simulink model "swift_6dof_sitl"  (R2026a)
settings: Solver=ode4  StopTime=inf  FixedStep=P.sitl.dt  MaxStep=0.01  RelTol=1e-6
InitFcn:
  | if ~evalin('base','exist(''P'',''var'')')
  |     evalin('base','swift_placeholder');
  | end
  | evalin('base','P = swift_sitl_params(P);');
StopFcn:
  | clear ap_json_step
undefined symbols (not defined in the file): P
libraries: aerolibasang x2, aerolibadyn x1, aerolibatmos2 x1
settings Model: Creator=rbilo  LastModifiedBy=Ryan

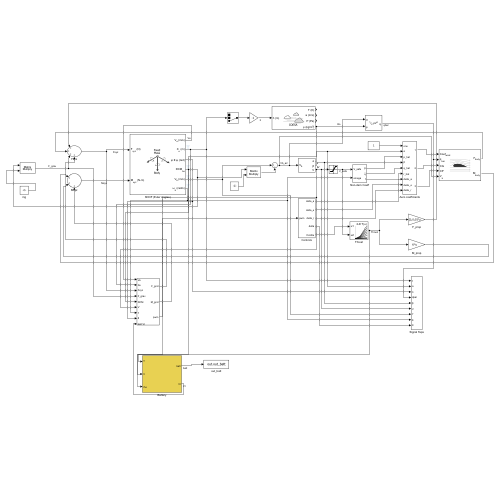
[thumbnail: Simulink's stored preview of the top-level diagram]
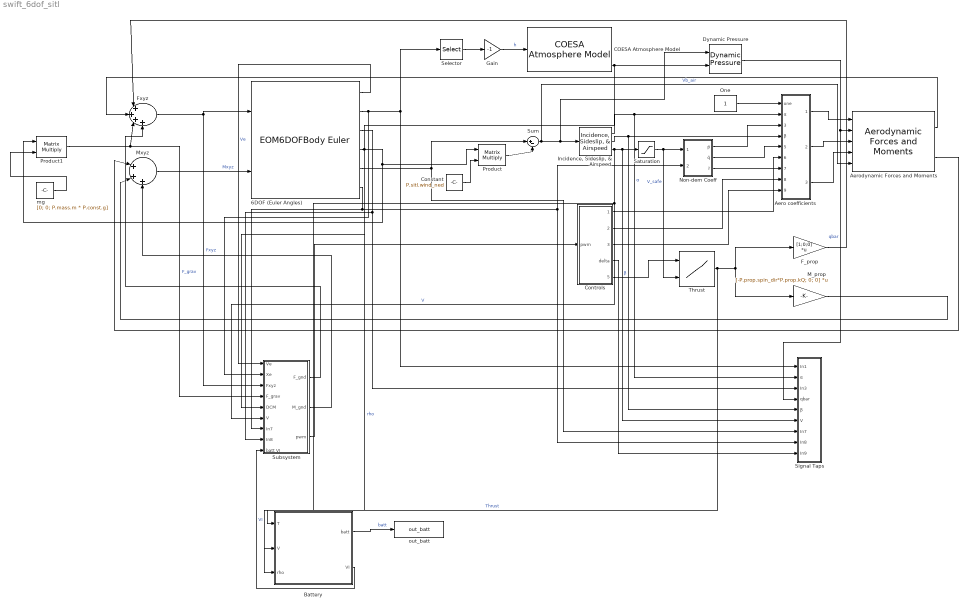
== system swift_6dof_sitl ==
  6DOF (Euler Angles) : EOM6DOFBodyEuler  xme_0=P.sitl.ic.pos0'  Vm_0=P.sitl.ic.uvw0'  eul_0=P.sitl.ic.euler0'  pm_0=P.sitl.ic.om0'  mass_0=P.mass.m  inertia=P.mass.I
  Aero coefficients : Subsystem
  "Aerodynamic Forces and Moments " : aerolibadyn/Aerodynamic Forces and Moments   inputAxes=Wind  outputForceAxes=Body  outputMomentAxes=Body  S=P.geom.S  b=P.geom.b  cbar=P.geom.c
  Battery : Subsystem
  COESA Atmosphere Model : aerolibatmos2/COESA Atmosphere Model  units=Metric (MKS)  spec=1976 COESA-extended U.S. Standard Atmosphere  model=Profile  profile_var=High temperature  profile_percent=1%  profile_alt=5 km (16404 ft)  envelope_var=High temperature  envelope_percent=1%  action=Warning
  Constant : Constant  Value=P.sitl.wind_ned
  Controls : Subsystem
  Dynamic Pressure : aerolibasang/Dynamic Pressure
  F_prop : Gain  Gain=[1;0;0]  Multiplication=Matrix(K*u)
  Fxyz : Sum  Inputs=|++++
  Gain : Gain  Gain=-1
  "Incidence, Sideslip, & Airspeed" : aerolibasang/Incidence, Sideslip, & Airspeed
  M_prop : Gain  Gain=[-P.prop.spin_dir*P.prop.kQ; 0; 0]  Multiplication=Matrix(K*u)
  Mxyz : Sum  Inputs=|+++
  Non-dem Coeff : Subsystem
  One : Constant
  Product : Product  Multiplication=Matrix(*)
  Product1 : Product  Multiplication=Matrix(*)
  Saturation : Saturate  UpperLimit=inf  LowerLimit=0.5
  Selector : Selector  InputPortWidth=3  IndexOptions=Index vector (dialog)  Indices=3  OutputSizes=1
  Signal Taps : Subsystem
  Subsystem : Subsystem
  Sum : Sum  Inputs=|+-
  Thrust : Lookup_n-D  BreakpointsForDimension1=P.prop.throttle_bp  BreakpointsForDimension2=P.prop.V_bp  Table=P.sitl.thrust_map  ExtrapMethod=Clip  InternalRulePriority=Speed  RndMeth=Simplest
      settings: InputPortMap=u0,u1
  mg : Constant  Value=[0; 0; P.mass.m * P.const.g]
  out_batt : ToWorkspace  VariableName=out_batt  SaveFormat=Timeseries  SampleTime=-1
      settings: Decimation=P.sitl.log_decim
  wires:
  6DOF (Euler Angles)/2 -> Subsystem/2(Xe), Signal Taps/1(In1), Selector/1
  6DOF (Euler Angles)/4 -> Subsystem/5(DCM), Product1/1, Product/1
  Constant/1 -> Product/2
  Selector/1 -> Gain/1
  Gain/1 -> COESA Atmosphere Model/1  "h"
  Product/1 -> Sum/2
  Sum/1 -> "Incidence, Sideslip, & Airspeed"/1, Dynamic Pressure/1, "Aerodynamic Forces and Moments "/5  "Vb_air"
  "Incidence, Sideslip, & Airspeed"/3 -> Subsystem/6(V), Battery/2(V), Signal Taps/6(V), Saturation/1  "V"
  COESA Atmosphere Model/4 -> Dynamic Pressure/2, Battery/3(rho)  "rho"
  Saturation/1 -> Thrust/2, Non-dem Coeff/1(V_safe)  "V_safe"
  6DOF (Euler Angles)/6 -> Subsystem/7(In7), Signal Taps/8(In8), Non-dem Coeff/2(omega)
  Dynamic Pressure/1 -> Signal Taps/4(qbar), "Aerodynamic Forces and Moments "/2  "qbar"
  "Incidence, Sideslip, & Airspeed"/1 -> Signal Taps/2(α), Aero coefficients/2(α)  "α"
  "Incidence, Sideslip, & Airspeed"/2 -> Signal Taps/5(β), Aero coefficients/4(β)  "β"
  Aero coefficients/1(Out1) -> "Aerodynamic Forces and Moments "/1
  Aero coefficients/2(Out2) -> "Aerodynamic Forces and Moments "/3
  Aero coefficients/3(Out3) -> "Aerodynamic Forces and Moments "/4
  One/1 -> Aero coefficients/1(one)
  Non-dem Coeff/1(p̂) -> Aero coefficients/3(p_hat)
  Non-dem Coeff/2(q̂) -> Aero coefficients/5(q_hat)
  Non-dem Coeff/3(r̂) -> Aero coefficients/6(r_hat)
  Controls/1(delta_a) -> Aero coefficients/7(delta_a)
  Controls/2(delta_e) -> Aero coefficients/8(delta_e)
  Controls/3(delta_r) -> Aero coefficients/9(delta_r)
  Controls/5(throttle) -> Thrust/1
  Thrust/1 -> F_prop/1, M_prop/1, Battery/1(T)  "Thrust"
  mg/1 -> Product1/2
  Product1/1 -> Subsystem/4(F_grav), Fxyz/3  "F_grav"
  Fxyz/1 -> Subsystem/3(Fxyz), 6DOF (Euler Angles)/1  "Fxyz"
  F_prop/1 -> Fxyz/1
  Mxyz/1 -> 6DOF (Euler Angles)/2  "Mxyz"
  M_prop/1 -> Mxyz/2
  "Aerodynamic Forces and Moments "/1 -> Fxyz/2
  "Aerodynamic Forces and Moments "/2 -> Mxyz/1
  6DOF (Euler Angles)/5 -> Signal Taps/7(In7), Sum/1
  6DOF (Euler Angles)/3 -> Subsystem/8(In8), Signal Taps/3(In3)
  Controls/4(delta) -> Signal Taps/9(In9)
  6DOF (Euler Angles)/1 -> Subsystem/1(Ve)  "Ve"
  Subsystem/1(F_gnd) -> Fxyz/4
  Subsystem/2(M_gnd) -> Mxyz/3
  Subsystem/3(pwm) -> Controls/1(pwm)
  Battery/1(batt) -> out_batt/1  "batt"
  Battery/2(VI) -> Subsystem/9(batt VI)  "VI"

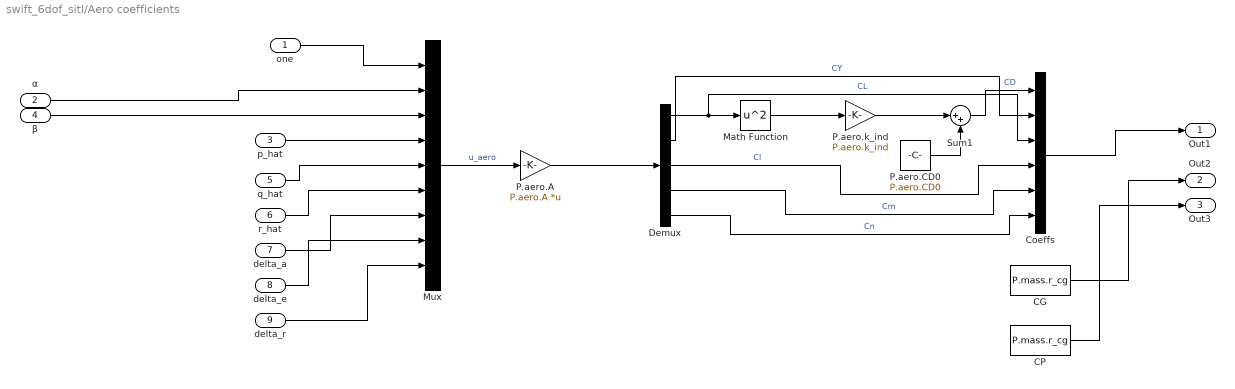
== system swift_6dof_sitl/Aero coefficients ==
  one : Inport
  α : Inport  Port=2
  p_hat : Inport  Port=3
  β : Inport  Port=4
  q_hat : Inport  Port=5
  r_hat : Inport  Port=6
  delta_a : Inport  Port=7
  delta_e : Inport  Port=8
  delta_r : Inport  Port=9
  CG : Constant  Value=P.mass.r_cg
  CP : Constant  Value=P.mass.r_cg
  Coeffs : Mux  Inputs=6
  Demux : Demux  Outputs=5
  Math Function : Math  Operator=square
  Mux : Mux  Inputs=9
  P.aero.A : Gain  Gain=P.aero.A  Multiplication=Matrix(K*u)
  P.aero.CD0 : Constant  Value=P.aero.CD0
  P.aero.k_ind : Gain  Gain=P.aero.k_ind
  Sum1 : Sum  Inputs=|++
  Out1 : Outport
  Out2 : Outport  Port=2
  Out3 : Outport  Port=3
  wires:
  P.aero.CD0/1 -> Sum1/2
  p_hat/1 -> Mux/4
  Demux/1 -> Math Function/1, Coeffs/3  "CL"
  delta_r/1 -> Mux/9
  Math Function/1 -> P.aero.k_ind/1
  CP/1 -> Out3/1
  P.aero.k_ind/1 -> Sum1/1
  P.aero.A/1 -> Demux/1
  delta_a/1 -> Mux/7
  Mux/1 -> P.aero.A/1  "u_aero"
  CG/1 -> Out2/1
  Demux/2 -> Coeffs/2  "CY"
  Sum1/1 -> Coeffs/1  "CD"
  β/1 -> Mux/3
  Demux/5 -> Coeffs/6  "Cn"
  Demux/3 -> Coeffs/4  "Cl"
  Demux/4 -> Coeffs/5  "Cm"
  r_hat/1 -> Mux/6
  Coeffs/1 -> Out1/1
  α/1 -> Mux/2
  q_hat/1 -> Mux/5
  one/1 -> Mux/1
  delta_e/1 -> Mux/8

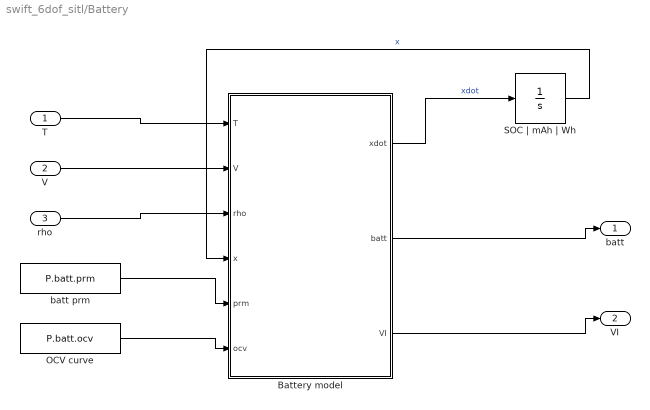
== system swift_6dof_sitl/Battery ==
  T : Inport
  V : Inport  Port=2
  rho : Inport  Port=3
  Battery model : MATLAB Function  TreatAsAtomicUnit=on
  OCV curve : Constant  Value=P.batt.ocv
  SOC | mAh | Wh : Integrator  InitialCondition=P.batt.x0  LimitOutput=on  UpperSaturationLimit=[1; inf; inf]  LowerSaturationLimit=[0; 0; 0]
  batt prm : Constant  Value=P.batt.prm
  batt : Outport
  VI : Outport  Port=2
  wires:
  T/1 -> Battery model/1(T)
  V/1 -> Battery model/2(V)
  rho/1 -> Battery model/3(rho)
  SOC | mAh | Wh/1 -> Battery model/4(x)  "x"
  batt prm/1 -> Battery model/5(prm)
  OCV curve/1 -> Battery model/6(ocv)
  Battery model/1(xdot) -> SOC | mAh | Wh/1  "xdot"
  Battery model/2(batt) -> batt/1
  Battery model/3(VI) -> VI/1

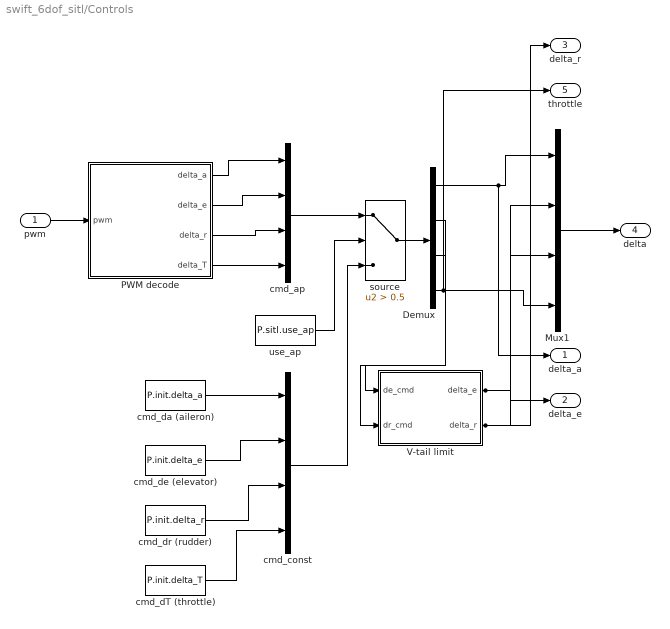
== system swift_6dof_sitl/Controls ==
  pwm : Inport
  Demux : Demux
  Mux1 : Mux
  PWM decode : Subsystem
  V-tail limit : Subsystem
  cmd_ap : Mux
  cmd_const : Mux
  cmd_dT (throttle) : Constant  Value=P.init.delta_T
  cmd_da (aileron) : Constant  Value=P.init.delta_a
  cmd_de (elevator) : Constant  Value=P.init.delta_e
  cmd_dr (rudder) : Constant  Value=P.init.delta_r
  source : Switch  Criteria=u2 > Threshold  Threshold=0.5  SaturateOnIntegerOverflow=off  InputSameDT=off
  use_ap : Constant  Value=P.sitl.use_ap
  delta_a : Outport
  delta_e : Outport  Port=2
  delta_r : Outport  Port=3
  delta : Outport  Port=4
  throttle : Outport  Port=5
  wires:
  pwm/1 -> PWM decode/1(pwm)
  use_ap/1 -> source/2
  PWM decode/1(delta_a) -> cmd_ap/1
  cmd_dr (rudder)/1 -> cmd_const/3
  cmd_da (aileron)/1 -> cmd_const/1
  cmd_de (elevator)/1 -> cmd_const/2
  PWM decode/2(delta_e) -> cmd_ap/2
  PWM decode/3(delta_r) -> cmd_ap/3
  PWM decode/4(delta_T) -> cmd_ap/4
  cmd_dT (throttle)/1 -> cmd_const/4
  cmd_ap/1 -> source/1
  cmd_const/1 -> source/3
  source/1 -> Demux/1
  Demux/1 -> delta_a/1, Mux1/1
  Demux/4 -> throttle/1, Mux1/4
  Mux1/1 -> delta/1
  Demux/2 -> V-tail limit/1(de_cmd)
  Demux/3 -> V-tail limit/2(dr_cmd)
  V-tail limit/1(delta_e) -> delta_e/1, Mux1/2
  V-tail limit/2(delta_r) -> delta_r/1, Mux1/3

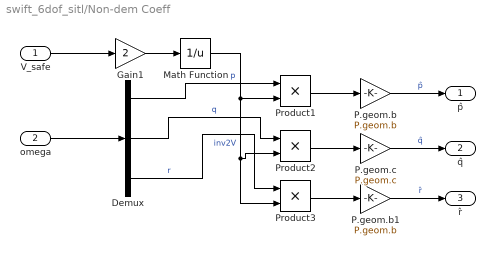
== system swift_6dof_sitl/Non-dem Coeff ==
  V_safe : Inport
  omega : Inport  Port=2
  Demux : Demux  Outputs=3
  Gain1 : Gain  Gain=2
  Math Function : Math  Operator=reciprocal
  P.geom.b : Gain  Gain=P.geom.b
  P.geom.b1 : Gain  Gain=P.geom.b
  P.geom.c : Gain  Gain=P.geom.c
  Product1 : Product
  Product2 : Product
  Product3 : Product
  p̂ : Outport
  q̂ : Outport  Port=2
  r̂ : Outport  Port=3
  wires:
  Math Function/1 -> Product2/2, Product3/2, Product1/2  "inv2V"
  Demux/2 -> Product2/1  "q"
  omega/1 -> Demux/1
  Product2/1 -> P.geom.c/1
  Demux/1 -> Product1/1  "p"
  Product1/1 -> P.geom.b/1
  Product3/1 -> P.geom.b1/1
  Gain1/1 -> Math Function/1
  Demux/3 -> Product3/1  "r"
  V_safe/1 -> Gain1/1
  P.geom.c/1 -> q̂/1  "q̂"
  P.geom.b/1 -> p̂/1  "p̂"
  P.geom.b1/1 -> r̂/1  "r̂"

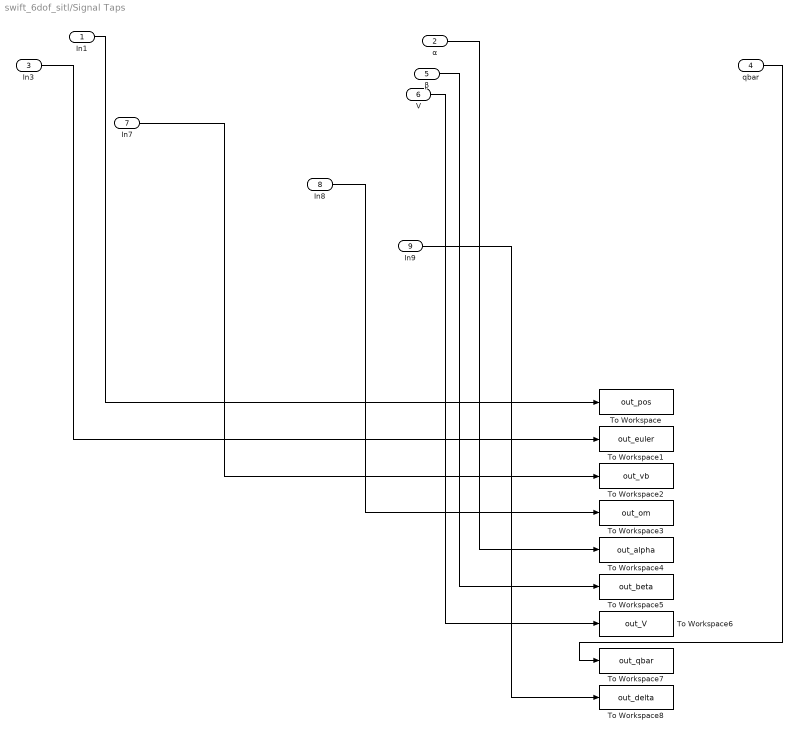
== system swift_6dof_sitl/Signal Taps ==
  In1 : Inport
  α : Inport  Port=2
  In3 : Inport  Port=3
  qbar : Inport  Port=4
  β : Inport  Port=5
  V : Inport  Port=6
  In7 : Inport  Port=7
  In8 : Inport  Port=8
  In9 : Inport  Port=9
  To Workspace : ToWorkspace  VariableName=out_pos  SaveFormat=Timeseries  SampleTime=-1
      settings: Decimation=P.sitl.log_decim
  To Workspace1 : ToWorkspace  VariableName=out_euler  SaveFormat=Timeseries  SampleTime=-1
      settings: Decimation=P.sitl.log_decim
  To Workspace2 : ToWorkspace  VariableName=out_vb  SaveFormat=Timeseries  SampleTime=-1
      settings: Decimation=P.sitl.log_decim
  To Workspace3 : ToWorkspace  VariableName=out_om  SaveFormat=Timeseries  SampleTime=-1
      settings: Decimation=P.sitl.log_decim
  To Workspace4 : ToWorkspace  VariableName=out_alpha  SaveFormat=Timeseries  SampleTime=-1
      settings: Decimation=P.sitl.log_decim
  To Workspace5 : ToWorkspace  VariableName=out_beta  SaveFormat=Timeseries  SampleTime=-1
      settings: Decimation=P.sitl.log_decim
  To Workspace6 : ToWorkspace  VariableName=out_V  SaveFormat=Timeseries  SampleTime=-1
      settings: Decimation=P.sitl.log_decim
  To Workspace7 : ToWorkspace  VariableName=out_qbar  SaveFormat=Timeseries  SampleTime=-1
      settings: Decimation=P.sitl.log_decim
  To Workspace8 : ToWorkspace  VariableName=out_delta  SaveFormat=Timeseries  SampleTime=-1
      settings: Decimation=P.sitl.log_decim
  wires:
  V/1 -> To Workspace6/1
  In3/1 -> To Workspace1/1
  α/1 -> To Workspace4/1
  qbar/1 -> To Workspace7/1
  β/1 -> To Workspace5/1
  In7/1 -> To Workspace2/1
  In9/1 -> To Workspace8/1
  In1/1 -> To Workspace/1
  In8/1 -> To Workspace3/1

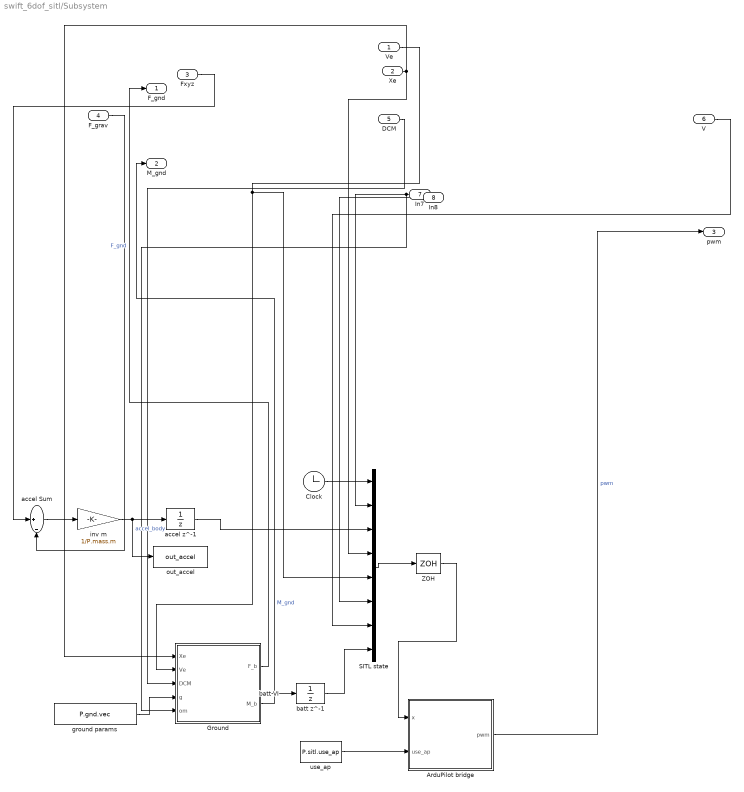
== system swift_6dof_sitl/Subsystem ==
  Ve : Inport
  Xe : Inport  Port=2
  Fxyz : Inport  Port=3
  F_grav : Inport  Port=4
  DCM : Inport  Port=5
  V : Inport  Port=6
  In7 : Inport  Port=7
  In8 : Inport  Port=8
  batt VI : Inport  Port=9
  ArduPilot bridge : MATLAB Function  TreatAsAtomicUnit=on
  Clock : Clock
  Ground : MATLAB Function  TreatAsAtomicUnit=on
  SITL state : Mux  Inputs=8
  ZOH : ZeroOrderHold  SampleTime=P.sitl.dt
  accel Sum : Sum  Inputs=|+-
  accel z^-1 : UnitDelay  InitialCondition=[0; 0; -P.const.g]  SampleTime=P.sitl.dt
  batt z^-1 : UnitDelay  InitialCondition=[P.batt.cells*interp1(P.batt.ocv(1,:), P.batt.ocv(2,:), P.batt.SOC0); 0]  SampleTime=P.sitl.dt
  ground params : Constant  Value=P.gnd.vec
  inv m : Gain  Gain=1/P.mass.m
  out_accel : ToWorkspace  VariableName=out_accel  SaveFormat=Timeseries  SampleTime=-1
      settings: Decimation=P.sitl.log_decim
  use_ap : Constant  Value=P.sitl.use_ap
  F_gnd : Outport
  M_gnd : Outport  Port=2
  pwm : Outport  Port=3
  wires:
  accel z^-1/1 -> SITL state/3
  inv m/1 -> accel z^-1/1, out_accel/1  "accel_body"
  use_ap/1 -> ArduPilot bridge/2(use_ap)
  ground params/1 -> Ground/4(g)
  Clock/1 -> SITL state/1
  Xe/1 -> SITL state/4, Ground/1(Xe)
  ZOH/1 -> ArduPilot bridge/1(x)
  SITL state/1 -> ZOH/1
  Ve/1 -> SITL state/5, Ground/2(Ve)
  accel Sum/1 -> inv m/1
  DCM/1 -> Ground/3(DCM)
  ArduPilot bridge/1(pwm) -> pwm/1  "pwm"
  Fxyz/1 -> accel Sum/1
  V/1 -> SITL state/7
  F_grav/1 -> accel Sum/2
  In8/1 -> SITL state/6
  In7/1 -> Ground/5(om), SITL state/2
  Ground/2(M_b) -> M_gnd/1  "M_gnd"
  Ground/1(F_b) -> F_gnd/1  "F_gnd"
  batt VI/1 -> batt z^-1/1
  batt z^-1/1 -> SITL state/8

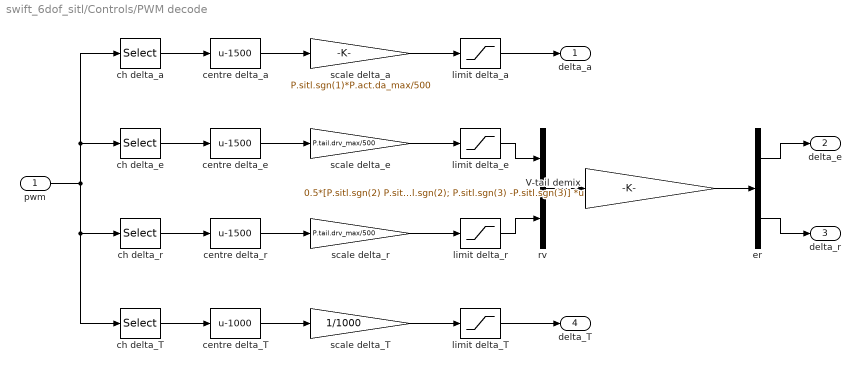
== system swift_6dof_sitl/Controls/PWM decode ==
  pwm : Inport
  V-tail demix : Gain  Gain=0.5*[P.sitl.sgn(2) P.sitl.sgn(2); P.sitl.sgn(3) -P.sitl.sgn(3)]  Multiplication=Matrix(K*u)
  centre delta_T : Bias  Bias=-1000  SaturateOnIntegerOverflow=off
  centre delta_a : Bias  Bias=-1500  SaturateOnIntegerOverflow=off
  centre delta_e : Bias  Bias=-1500  SaturateOnIntegerOverflow=off
  centre delta_r : Bias  Bias=-1500  SaturateOnIntegerOverflow=off
  ch delta_T : Selector  InputPortWidth=16  IndexOptions=Index vector (dialog)  Indices=P.sitl.ch(4)  OutputSizes=1
  ch delta_a : Selector  InputPortWidth=16  IndexOptions=Index vector (dialog)  Indices=P.sitl.ch(1)  OutputSizes=1
  ch delta_e : Selector  InputPortWidth=16  IndexOptions=Index vector (dialog)  Indices=P.sitl.ch(2)  OutputSizes=1
  ch delta_r : Selector  InputPortWidth=16  IndexOptions=Index vector (dialog)  Indices=P.sitl.ch(3)  OutputSizes=1
  er : Demux  Outputs=2
  limit delta_T : Saturate  UpperLimit=1  LowerLimit=0
  limit delta_a : Saturate  UpperLimit=P.act.da_max  LowerLimit=-P.act.da_max
  limit delta_e : Saturate  UpperLimit=P.tail.drv_max  LowerLimit=-P.tail.drv_max
  limit delta_r : Saturate  UpperLimit=P.tail.drv_max  LowerLimit=-P.tail.drv_max
  rv : Mux  Inputs=2
  scale delta_T : Gain  Gain=1/1000
  scale delta_a : Gain  Gain=P.sitl.sgn(1)*P.act.da_max/500
  scale delta_e : Gain  Gain=P.tail.drv_max/500
  scale delta_r : Gain  Gain=P.tail.drv_max/500
  delta_a : Outport
  delta_e : Outport  Port=2
  delta_r : Outport  Port=3
  delta_T : Outport  Port=4
  wires:
  pwm/1 -> ch delta_r/1, ch delta_T/1, ch delta_a/1, ch delta_e/1
  ch delta_a/1 -> centre delta_a/1
  centre delta_a/1 -> scale delta_a/1
  scale delta_a/1 -> limit delta_a/1
  limit delta_a/1 -> delta_a/1
  ch delta_e/1 -> centre delta_e/1
  centre delta_e/1 -> scale delta_e/1
  scale delta_e/1 -> limit delta_e/1
  ch delta_r/1 -> centre delta_r/1
  centre delta_r/1 -> scale delta_r/1
  scale delta_r/1 -> limit delta_r/1
  ch delta_T/1 -> centre delta_T/1
  centre delta_T/1 -> scale delta_T/1
  scale delta_T/1 -> limit delta_T/1
  limit delta_T/1 -> delta_T/1
  limit delta_e/1 -> rv/1
  limit delta_r/1 -> rv/2
  rv/1 -> V-tail demix/1
  V-tail demix/1 -> er/1
  er/1 -> delta_e/1
  er/2 -> delta_r/1

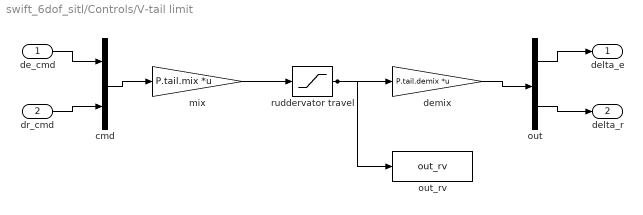
== system swift_6dof_sitl/Controls/V-tail limit ==
  de_cmd : Inport
  dr_cmd : Inport  Port=2
  cmd : Mux  Inputs=2
  demix : Gain  Gain=P.tail.demix  Multiplication=Matrix(K*u)
  mix : Gain  Gain=P.tail.mix  Multiplication=Matrix(K*u)
  out : Demux  Outputs=2
  out_rv : ToWorkspace  VariableName=out_rv  SaveFormat=Timeseries  SampleTime=-1
      settings: Decimation=P.sitl.log_decim
  ruddervator travel : Saturate  UpperLimit=P.tail.drv_max  LowerLimit=-P.tail.drv_max
  delta_e : Outport
  delta_r : Outport  Port=2
  wires:
  de_cmd/1 -> cmd/1
  dr_cmd/1 -> cmd/2
  cmd/1 -> mix/1
  mix/1 -> ruddervator travel/1
  ruddervator travel/1 -> demix/1, out_rv/1
  demix/1 -> out/1
  out/1 -> delta_e/1
  out/2 -> delta_r/1

== matlab function swift_6dof_sitl/Subsystem/Ground ==
  data: Xe input; F_b output; Ve input; DCM input; g input; om input; M_b output
function [F_b, M_b] = ground(Xe, Ve, DCM, g, om)
%GROUND v2  Three-wheel spring-damper runway with friction (stage 3b).
%   Xe  NED position (m)      Ve  NED velocity (m/s)
%   DCM NED -> body            om  body rates (rad/s)
%   g = [on; k; c; mu_roll; mu_lat; v_eps; wheels(:)]   (15 x 1)
%   F_b, M_b  wheel forces and moments about the CG, body axes.
F_b = zeros(3,1);
M_b = zeros(3,1);
if g(1) < 0.5
    return
end
k = g(2);  c = g(3);  mur = g(4);  mul = g(5);  ve = max(g(6), 1e-3);
R   = reshape(g(7:15), 3, 3);       % wheel contact points, body axes
Cbe = DCM';                         % body -> NED
xh  = [Cbe(1,1); Cbe(2,1); 0];       % nose direction along the runway
n   = sqrt(xh(1)^2 + xh(2)^2);
if n < 1e-6
    xh = [1; 0; 0];
else
    xh = xh / n;
end
yh = [-xh(2); xh(1); 0];             % right wing direction along the runway
for i = 1:3
    r   = R(:, i);
    p   = Xe + Cbe * r;              % wheel position, NED
    if p(3) > 0                      % below the runway surface
        v = Ve + Cbe * cross(om, r); % wheel velocity, NED
        N = k * p(3) + c * v(3);     % normal load, N
        if N > 0
            vl = xh' * v;
            vs = yh' * v;
            F  = [0; 0; -N] - mur*N*tanh(vl/ve)*xh - mul*N*tanh(vs/ve)*yh;
            Fb = DCM * F;
            F_b = F_b + Fb;
            M_b = M_b + cross(r, Fb);
        end
    end
end

== matlab function swift_6dof_sitl/Subsystem/ArduPilot bridge ==
  settings: updateMethod=DISCRETE  sampleTime=P.sitl.dt
  data: x input; pwm output; use_ap input
function pwm = bridge(x, use_ap)
%BRIDGE  ArduPilot JSON SITL, one frame per fixed step (guide steps 10 + 13).
%   x = [t; gyro(3); accel_body(3); pos(3); vel(3); euler(3); airspeed]
%   use_ap = 0 skips the network entirely and returns neutral PWM.
coder.extrinsic('ap_json_step');
pwm = [1500; 1500; 1000; 1500; 1500*ones(12,1)];
if use_ap > 0.5
    pwm = ap_json_step(x);
end

== matlab function swift_6dof_sitl/Battery/Battery model ==
  data: T input; xdot output; V input; rho input; x input; prm input; ocv input; batt output; VI output
function [xdot, batt, VI] = battery(T, V, rho, x, prm, ocv)
%BATTERY  SWIFT battery model. All the physics is in swift_battery_fcn.m.
%   T N, V m/s, rho kg/m^3, x = [SOC; mAh; Wh], prm = P.batt.prm, ocv = P.batt.ocv
[xdot, batt, VI] = swift_battery_fcn(T, V, rho, x, prm, ocv);
